simulink model "lab3_poles"  (R2025b)
settings: Solver=ode45  StartTime=0.0  StopTime=10  MaxStep=0.02  RelTol=1e-3
libraries: simulink x1
settings Model: Creator=Nickolay  LastModifiedBy=Nickolay

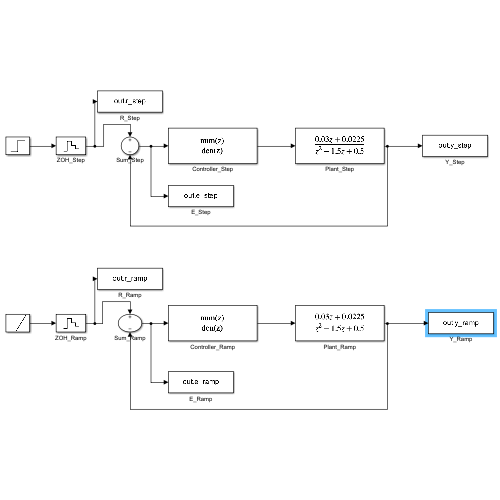
[thumbnail: Simulink's stored preview of the top-level diagram]
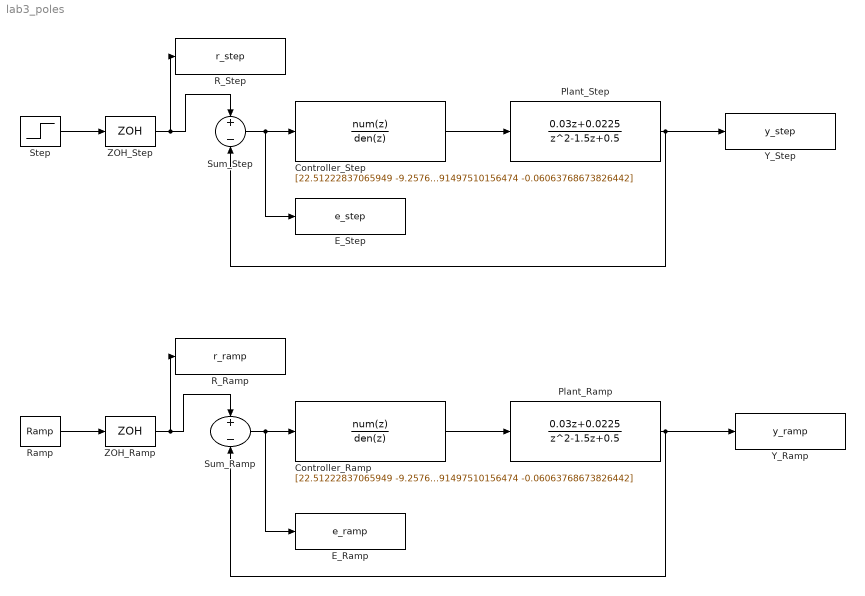
== system lab3_poles ==
  Controller_Ramp : DiscreteTransferFcn  Numerator=[22.51222837065949 -9.25768252890531 -0.9992158282122188]  Denominator=[1 0.6691497510156474 -0.06063768673826442]  SampleTime=0.2
  Controller_Step : DiscreteTransferFcn  Numerator=[22.51222837065949 -9.25768252890531 -0.9992158282122188]  Denominator=[1 0.6691497510156474 -0.06063768673826442]  SampleTime=0.2
  E_Ramp : ToWorkspace  VariableName=e_ramp  SaveFormat=Timeseries  SampleTime=-1
  E_Step : ToWorkspace  VariableName=e_step  SaveFormat=Timeseries  SampleTime=-1
  Plant_Ramp : DiscreteTransferFcn  Numerator=[0.03 0.0225]  Denominator=[1 -1.5 0.5]  SampleTime=0.2
  Plant_Step : DiscreteTransferFcn  Numerator=[0.03 0.0225]  Denominator=[1 -1.5 0.5]  SampleTime=0.2
  R_Ramp : ToWorkspace  VariableName=r_ramp  SaveFormat=Timeseries  SampleTime=-1
  R_Step : ToWorkspace  VariableName=r_step  SaveFormat=Timeseries  SampleTime=-1
  Ramp : simulink/Sources/Ramp  slope=1  start=0  InitialOutput=0
  Step : Step  Time=0  SampleTime=0.2
  Sum_Ramp : Sum  Inputs=+-
  Sum_Step : Sum  Inputs=+-
  Y_Ramp : ToWorkspace  VariableName=y_ramp  SaveFormat=Timeseries  SampleTime=-1
  Y_Step : ToWorkspace  VariableName=y_step  SaveFormat=Timeseries  SampleTime=-1
  ZOH_Ramp : ZeroOrderHold  SampleTime=0.2
  ZOH_Step : ZeroOrderHold  SampleTime=0.2
  wires:
  Step/1 -> ZOH_Step/1
  ZOH_Step/1 -> Sum_Step/1, R_Step/1
  Sum_Step/1 -> E_Step/1, Controller_Step/1
  Controller_Step/1 -> Plant_Step/1
  Plant_Step/1 -> Sum_Step/2, Y_Step/1
  Ramp/1 -> ZOH_Ramp/1
  ZOH_Ramp/1 -> Sum_Ramp/1, R_Ramp/1
  Sum_Ramp/1 -> E_Ramp/1, Controller_Ramp/1
  Controller_Ramp/1 -> Plant_Ramp/1
  Plant_Ramp/1 -> Sum_Ramp/2, Y_Ramp/1
